simulink model "part1_dc_motor_linearization"  (R2024b)
settings: Solver=ode45  StartTime=0.0  StopTime=2  MaxStep=0.002  RelTol=1e-8  AbsTol=1e-10
model workspace (MAT data in the model file):
  J = 0.01
  KT = 0.2
  Ke = 0.2
  La = 0.05
  Ra = 2
  d1 = 0.01
  d2 = 0.005
  ia0 = 0
  omega0 = 0
  theta0 = 0
settings Model: Creator=matiasgarcia  LastModifiedBy=matiasgarcia
settings DataIOCC: SaveOutput=off  SignalLogging=off  SaveTime=off

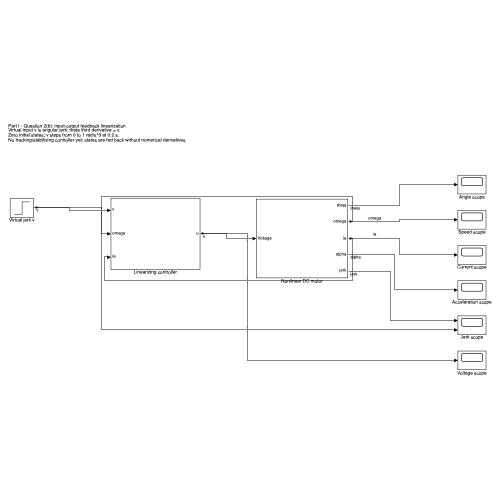
[thumbnail: Simulink's stored preview of the top-level diagram]
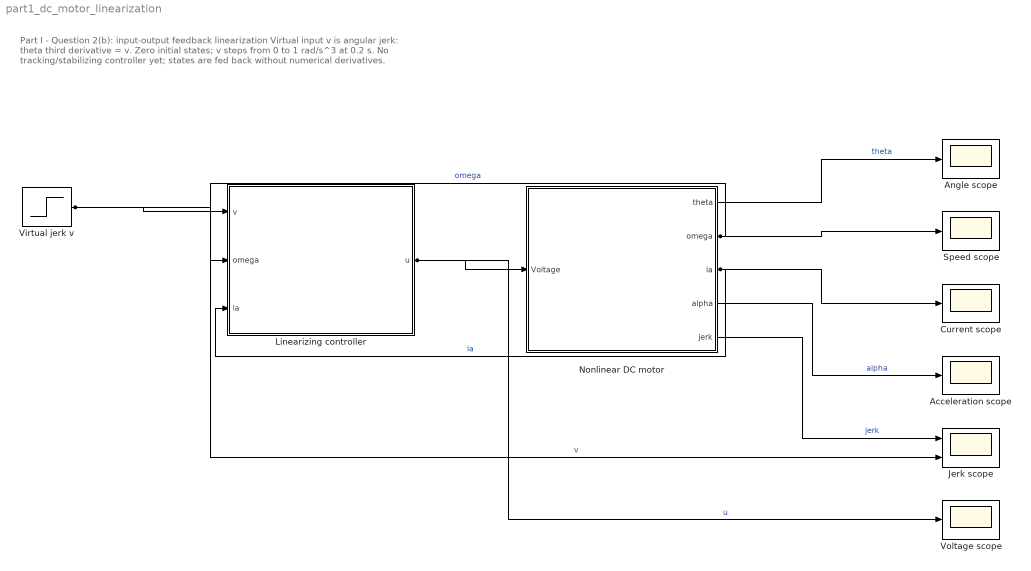
== system part1_dc_motor_linearization ==
  note: Part I - Question 2(b): input-output feedback linearization
      | Virtual input v is angular jerk: theta third derivative = v.
      | Zero initial states; v steps from 0 to 1 rad/s^3 at 0.2 s.
      | No tracking/stabilizing controller yet; states are fed back without numerical derivatives.
  Acceleration scope : Scope
  Angle scope : Scope
  Current scope : Scope
  Jerk scope : Scope  NumInputPorts=2
  Linearizing controller : Subsystem
  Nonlinear DC motor : Subsystem
  Speed scope : Scope
  Virtual jerk v : Step  Time=0.2  SampleTime=0
  Voltage scope : Scope
  wires:
  Nonlinear DC motor/1(theta) -> Angle scope/1  "theta"
  Nonlinear DC motor/2(omega) -> Speed scope/1, Linearizing controller/2(omega)  "omega"
  Nonlinear DC motor/3(ia) -> Current scope/1, Linearizing controller/3(ia)  "ia"
  Nonlinear DC motor/4(alpha) -> Acceleration scope/1  "alpha"
  Nonlinear DC motor/5(jerk) -> Jerk scope/1  "jerk"
  Virtual jerk v/1 -> Linearizing controller/1(v), Jerk scope/2  "v"
  Linearizing controller/1(u) -> Nonlinear DC motor/1(Voltage), Voltage scope/1  "u"

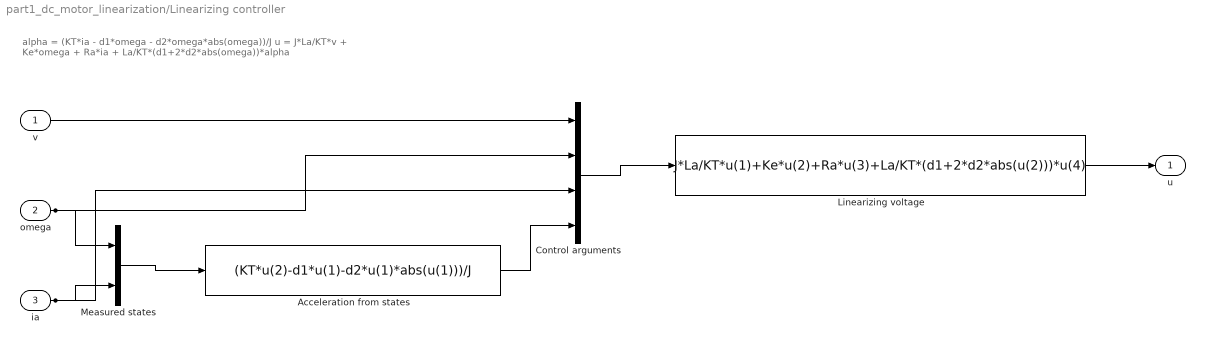
== system part1_dc_motor_linearization/Linearizing controller ==
  note: alpha = (KT*ia - d1*omega - d2*omega*abs(omega))/J
      | u = J*La/KT*v + Ke*omega + Ra*ia + La/KT*(d1+2*d2*abs(omega))*alpha
  v : Inport
  omega : Inport  Port=2
  ia : Inport  Port=3
  Acceleration from states : Fcn  Expr=(KT*u(2)-d1*u(1)-d2*u(1)*abs(u(1)))/J
  Control arguments : Mux
  Linearizing voltage : Fcn  Expr=J*La/KT*u(1)+Ke*u(2)+Ra*u(3)+La/KT*(d1+2*d2*abs(u(2)))*u(4)
  Measured states : Mux  Inputs=2
  u : Outport
  wires:
  omega/1 -> Measured states/1, Control arguments/2
  ia/1 -> Measured states/2, Control arguments/3
  Measured states/1 -> Acceleration from states/1
  v/1 -> Control arguments/1
  Acceleration from states/1 -> Control arguments/4
  Control arguments/1 -> Linearizing voltage/1
  Linearizing voltage/1 -> u/1

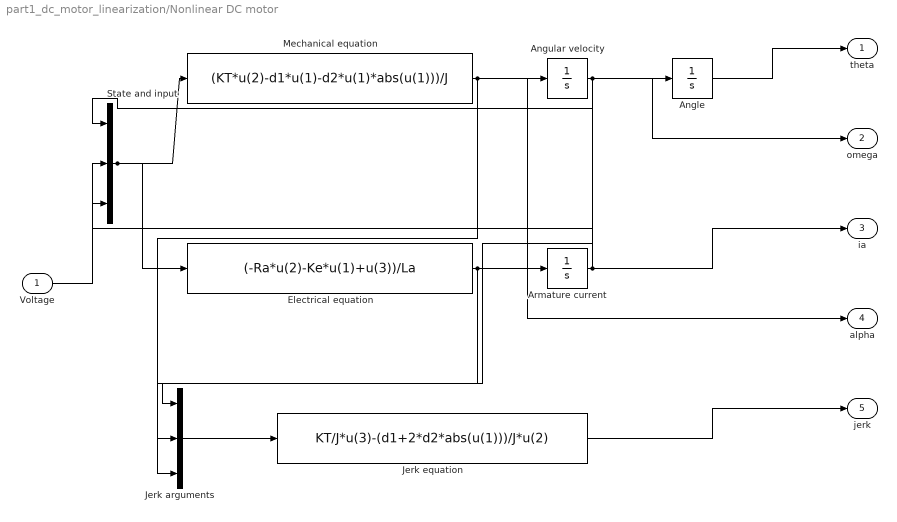
== system part1_dc_motor_linearization/Nonlinear DC motor ==
  Voltage : Inport
  Angle : Integrator  InitialCondition=theta0
  Angular velocity : Integrator  InitialCondition=omega0
  Armature current : Integrator  InitialCondition=ia0
  Electrical equation : Fcn  Expr=(-Ra*u(2)-Ke*u(1)+u(3))/La
  Jerk arguments : Mux  Inputs=3
  Jerk equation : Fcn  Expr=KT/J*u(3)-(d1+2*d2*abs(u(1)))/J*u(2)
  Mechanical equation : Fcn  Expr=(KT*u(2)-d1*u(1)-d2*u(1)*abs(u(1)))/J
  State and input : Mux  Inputs=3
  theta : Outport
  omega : Outport  Port=2
  ia : Outport  Port=3
  alpha : Outport  Port=4
  jerk : Outport  Port=5
  wires:
  Angular velocity/1 -> State and input/1, Angle/1, Jerk arguments/1, omega/1
  Armature current/1 -> State and input/2, ia/1
  Voltage/1 -> State and input/3
  State and input/1 -> Mechanical equation/1, Electrical equation/1
  Mechanical equation/1 -> Angular velocity/1, Jerk arguments/2, alpha/1
  Electrical equation/1 -> Armature current/1, Jerk arguments/3
  Jerk arguments/1 -> Jerk equation/1
  Angle/1 -> theta/1
  Jerk equation/1 -> jerk/1
